simulink model "chaine_qpsk_cod"  (R2026b)
settings: Solver=FixedStepDiscrete  StopTime=1000  FixedStep=1/7
values from neighbouring files (symbols this model uses):
  graine = round(P.graine)    [Parametres.m]    (also in Partie2.m = P.graine; parametres_perso.m = mod(sum(c .* (1:numel(c)) * 31) + 7 * numel(c), 2^31 - 1))
  sig2 = 0.25/EbN0    [test_qpsk.m]    (also in test_qpsk_cod.m = (7/16)/EbN0)
libraries: simulink x1
settings Model: Creator=INS NAWEL  LastModifiedBy=INS NAWEL

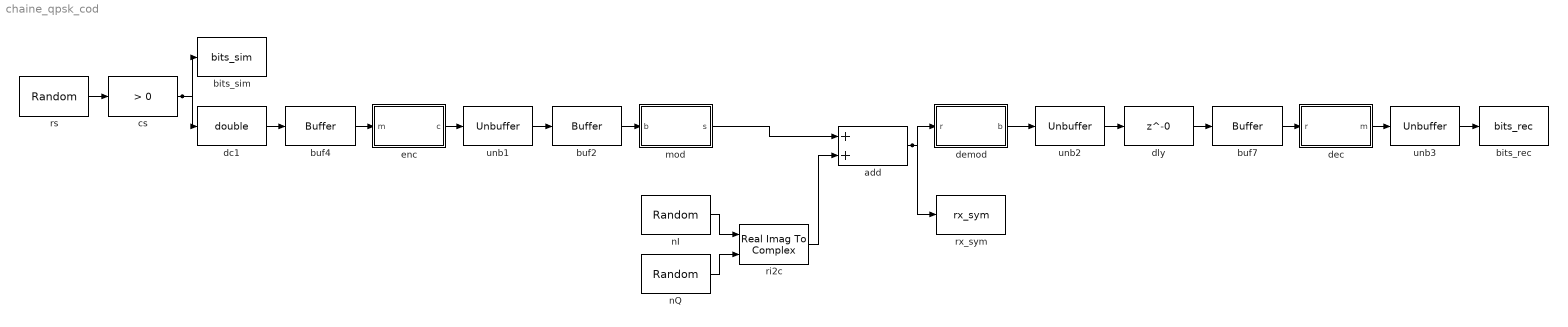
== system chaine_qpsk_cod ==
  add : Sum
  bits_rec : ToWorkspace  VariableName=bits_rec  SampleTime=1
  bits_sim : ToWorkspace  VariableName=bits_sim  SampleTime=1
  buf2 : Buffer  N=2
  buf4 : Buffer  N=4
  buf7 : Buffer  N=7
  cs : simulink/Logic and Bit Operations/Compare To Constant  relop=>  const=0  OutDataTypeStr=boolean
  dc1 : DataTypeConversion  OutDataTypeStr=double  SaturateOnIntegerOverflow=off  RndMeth=Floor
  dec : MATLAB Function  TreatAsAtomicUnit=on
  demod : MATLAB Function  TreatAsAtomicUnit=on
  dly : Delay  DelayLength=0
  enc : MATLAB Function  TreatAsAtomicUnit=on
  mod : MATLAB Function  TreatAsAtomicUnit=on
  nI : RandomNumber  Variance=sig2  Seed=graine+2  SampleTime=8/7
  nQ : RandomNumber  Variance=sig2  Seed=graine+3  SampleTime=8/7
  ri2c : RealImagToComplex
  rs : RandomNumber  Seed=graine+1  SampleTime=1
  rx_sym : ToWorkspace  VariableName=rx_sym  SampleTime=8/7
  unb1 : Unbuffer
  unb2 : Unbuffer
  unb3 : Unbuffer
  wires:
  rs/1 -> cs/1
  cs/1 -> bits_sim/1, dc1/1
  dc1/1 -> buf4/1
  buf4/1 -> enc/1(m)
  enc/1(c) -> unb1/1
  unb1/1 -> buf2/1
  buf2/1 -> mod/1(b)
  mod/1(s) -> add/1
  nI/1 -> ri2c/1
  nQ/1 -> ri2c/2
  ri2c/1 -> add/2
  add/1 -> rx_sym/1, demod/1(r)
  demod/1(b) -> unb2/1
  unb2/1 -> dly/1
  dly/1 -> buf7/1
  buf7/1 -> dec/1(r)
  dec/1(m) -> unb3/1
  unb3/1 -> bits_rec/1

== matlab function chaine_qpsk_cod/enc ==
  data: m input; c output
function c = enc(m)
%#codegen
P = [1 1 0; 0 1 1; 1 1 1; 1 0 1];
G = [eye(4) P];
c = mod(G'*double(m(:)), 2);
end

== matlab function chaine_qpsk_cod/demod ==
  data: r input; b output
function b = qpsk_demod(r)
%#codegen
b = [double(real(r) < 0); double(imag(r) < 0)];
end

== matlab function chaine_qpsk_cod/dec ==
  data: r input; m output
function m = dec(r)
%#codegen
P = [1 1 0; 0 1 1; 1 1 1; 1 0 1];
H = [P' eye(3)];
x = double(r(:));
s = mod(H*x, 2);
idx = s(1) + 2*s(2) + 4*s(3);
pos = [5 6 1 7 4 2 3];
if idx > 0
    j = pos(idx);
    x(j) = 1 - x(j);
end
m = x(1:4);
end

== matlab function chaine_qpsk_cod/mod ==
  data: b input; s output
function s = qpsk_mod(b)
%#codegen
b = double(b(:));
s = ((1-2*b(1)) + 1j*(1-2*b(2)))/sqrt(2);
end
